simulink model "adder_04_c"  (R2026b)
settings: Solver=FixedStepDiscrete  StartTime=0  StopTime=0.5  FixedStep=0.01
model workspace (MAT data in the model file):
  loop_gain = Simulink.Parameter
  loop_gain.Value = 1
  loop_gain.Complexity = 'real'
  loop_gain.Dimensions = [1 1]
settings Model: ParameterArgumentNames=loop_gain  Creator=Fasih  LastModifiedBy=Fasih

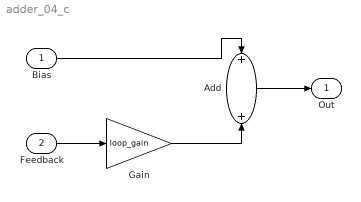
== system adder_04_c ==
  Bias : Inport
  Feedback : Inport  Port=2
  Add : Sum
  Gain : Gain  Gain=loop_gain
  Out : Outport
  wires:
  Bias/1 -> Add/1
  Feedback/1 -> Gain/1
  Gain/1 -> Add/2
  Add/1 -> Out/1
